simulink model "bench_local_2208"  (R2026a)
settings: Solver=FixedStepDiscrete  StopTime=bench_duration  FixedStep=Ts_plant
model workspace (MAT data in the model file):
  B_load = 0
  B_m = 0.00357610067176
  B_rotor = 1.07e-06
  IQ_LIMIT_MA = 400
  I_console_max_mA = 1800
  Imax = 200
  J_load = 0
  J_m = 5e-07
  J_rotor = 5e-07
  Ke_LL_rms_per_krpm = 7.68
  Ki_i = 0.0008
  Ki_w = 200
  Kp_i = 0.00025
  Kp_w = 27
  L_d = 0.00258
  L_q = 0.00258
  MAX_FILTERED_SPEED = 35
  MAX_PHASE_MA = 800
  MAX_RAW_SPEED = 60
  MOD_LIMIT = 0.12
  R_s = 9.21741944903
  R_shunt = 0.015
  STUCK_CHECK_MOD = 0.02
  STUCK_CHECK_US = 120000
  Ts_ctrl = 0.001
  Ts_plant = 1e-05
  V_dc = 12
  adc_bits = 12
  adc_range_mV = 3100
  alpha_i = 0.15
  alpha_w = 0.05
  b_u_mV = 1680
  b_v_mV = 1680
  bench_amp = 2
  bench_duration = 5
  bench_hz = 1
  bench_speed = 1
  ctrl_dt_max_s = 0.05
  duty_mid = 0.5
  enc_bits = 12
  enc_dt_max_us = 20000
  enc_dt_min_us = 100
  enc_fail_decay = 0.9
  enc_ok = 1
  f_closed_max_Hz = 60
  f_console_max_Hz = 80
  id_target_mA = 0
  load_Nm = 0.002
  mod_limit = 0.4
  motor_x0 = [0; 0; 0; 0]
  ocp_disable_s = 0.02
  ocp_limit_mA = 1500
  ocp_samples = 150
  p_pairs = 7
  psi_pm = 0.00855438776211
  pwm_Hz = 20000
  pwm_bits = 10
  pwm_switching = 0
  restoring_A_per_rad = 1.99244538017
  s_enc = 1
  sense_gain = 50
  sense_sign = -1
  sense_wiring_sign = -1
  sim_end_s = 3
  start_Hz = 0
  start_load_Nm = 0
  step_load_s = 1.25
  step_speed_s = 0.1
  target_Hz = 8
  theta_off = 0
  torque_sign = 1
  unipolar_threshold_mV = 300
Description:
  | BENCH1 small-angle experiment. Model Workspace owns the complete parameter snapshot. R_s (ohm), B_m (N m s/rad), restoring_A_per_rad (A/rad) specify the local plant. Set bench_speed=1 for electrical speed, 0 for q current; bench_hz is the reference frequency and bench_amp is its peak in electrical rad/s or mA.
settings Model: Creator=29113  LastModifiedBy=29113

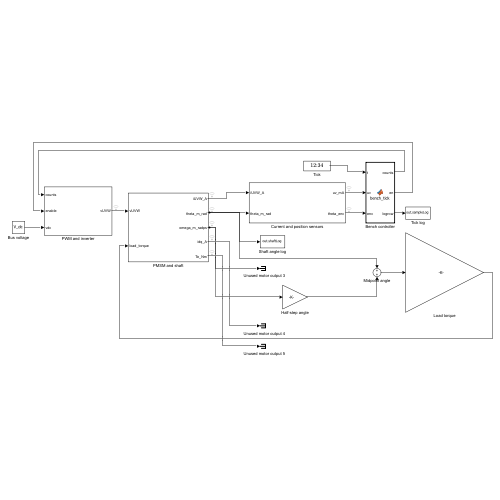
[thumbnail: Simulink's stored preview of the top-level diagram]
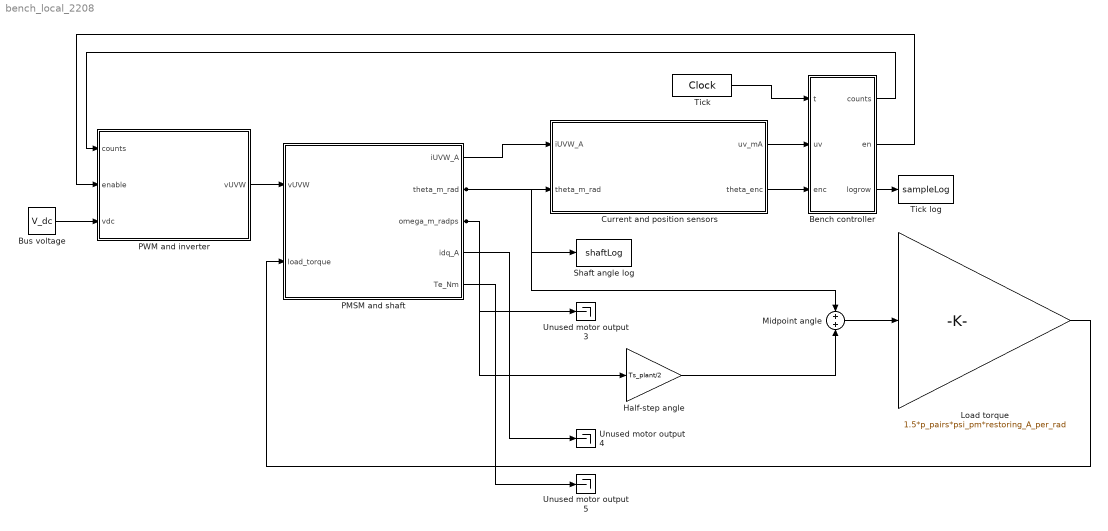
== system bench_local_2208 ==
  Bench controller : MATLAB Function  TreatAsAtomicUnit=on
  Bus voltage : Constant  Value=V_dc  SampleTime=Ts_plant
  Current and position sensors : Subsystem
  Half-step angle : Gain  Gain=Ts_plant/2
  Load torque : Gain  Gain=1.5*p_pairs*psi_pm*restoring_A_per_rad
  Midpoint angle : Sum
  PMSM and shaft : Subsystem
  PWM and inverter : Subsystem
  Shaft angle log : ToWorkspace  VariableName=shaftLog  SaveFormat=Timeseries  SampleTime=Ts_ctrl
  Tick : DigitalClock  SampleTime=Ts_ctrl
  Tick log : ToWorkspace  VariableName=sampleLog  SaveFormat=Timeseries  SampleTime=-1
  Unused motor output 3 : Terminator
  Unused motor output 4 : Terminator
  Unused motor output 5 : Terminator
  wires:
  Bus voltage/1 -> PWM and inverter/3(vdc)
  PMSM and shaft/4(idq_A) -> Unused motor output 4/1
  PWM and inverter/1(vUVW) -> PMSM and shaft/1(vUVW)
  PMSM and shaft/1(iUVW_A) -> Current and position sensors/1(iUVW_A)
  PMSM and shaft/2(theta_m_rad) -> Midpoint angle/1, Current and position sensors/2(theta_m_rad), Shaft angle log/1
  PMSM and shaft/5(Te_Nm) -> Unused motor output 5/1
  PMSM and shaft/3(omega_m_radps) -> Half-step angle/1, Unused motor output 3/1
  Midpoint angle/1 -> Load torque/1
  Tick/1 -> Bench controller/1(t)
  Bench controller/2(en) -> PWM and inverter/2(enable)
  Current and position sensors/1(uv_mA) -> Bench controller/2(uv)
  Current and position sensors/2(theta_enc) -> Bench controller/3(enc)
  Half-step angle/1 -> Midpoint angle/2
  Bench controller/1(counts) -> PWM and inverter/1(counts)
  Bench controller/3(logrow) -> Tick log/1
  Load torque/1 -> PMSM and shaft/2(load_torque)

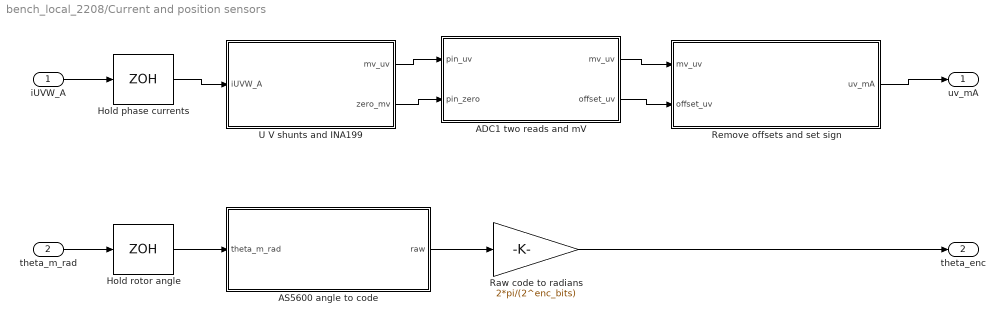
== system bench_local_2208/Current and position sensors ==
  iUVW_A : Inport
  theta_m_rad : Inport  Port=2
  ADC1 two reads and mV : MATLAB Function  TreatAsAtomicUnit=on
  AS5600 angle to code : MATLAB Function  TreatAsAtomicUnit=on
  Hold phase currents : ZeroOrderHold  SampleTime=Ts_ctrl
  Hold rotor angle : ZeroOrderHold  SampleTime=Ts_ctrl
  Raw code to radians : Gain  Gain=2*pi/(2^enc_bits)
  Remove offsets and set sign : MATLAB Function  TreatAsAtomicUnit=on
  U V shunts and INA199 : MATLAB Function  TreatAsAtomicUnit=on
  uv_mA : Outport
  theta_enc : Outport  Port=2
  wires:
  Raw code to radians/1 -> theta_enc/1
  AS5600 angle to code/1(raw) -> Raw code to radians/1
  Hold rotor angle/1 -> AS5600 angle to code/1(theta_m_rad)
  theta_m_rad/1 -> Hold rotor angle/1
  Remove offsets and set sign/1(uv_mA) -> uv_mA/1
  ADC1 two reads and mV/2(offset_uv) -> Remove offsets and set sign/2(offset_uv)
  ADC1 two reads and mV/1(mv_uv) -> Remove offsets and set sign/1(mv_uv)
  U V shunts and INA199/2(zero_mv) -> ADC1 two reads and mV/2(pin_zero)
  U V shunts and INA199/1(mv_uv) -> ADC1 two reads and mV/1(pin_uv)
  Hold phase currents/1 -> U V shunts and INA199/1(iUVW_A)
  iUVW_A/1 -> Hold phase currents/1

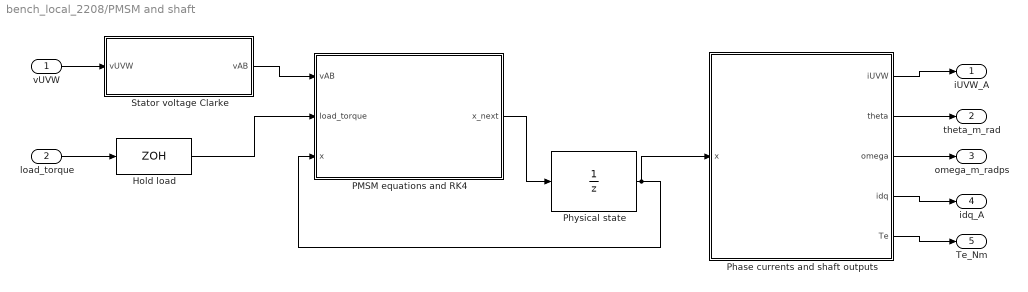
== system bench_local_2208/PMSM and shaft ==
  vUVW : Inport
  load_torque : Inport  Port=2
  Hold load : ZeroOrderHold  SampleTime=Ts_plant
  PMSM equations and RK4 : MATLAB Function  TreatAsAtomicUnit=on
  Phase currents and shaft outputs : MATLAB Function  TreatAsAtomicUnit=on
  Physical state : UnitDelay  InitialCondition=motor_x0  SampleTime=Ts_plant
  Stator voltage Clarke : MATLAB Function  TreatAsAtomicUnit=on
  iUVW_A : Outport
  theta_m_rad : Outport  Port=2
  omega_m_radps : Outport  Port=3
  idq_A : Outport  Port=4
  Te_Nm : Outport  Port=5
  wires:
  PMSM equations and RK4/1(x_next) -> Physical state/1
  Physical state/1 -> Phase currents and shaft outputs/1(x), PMSM equations and RK4/3(x)
  Hold load/1 -> PMSM equations and RK4/2(load_torque)
  load_torque/1 -> Hold load/1
  Stator voltage Clarke/1(vAB) -> PMSM equations and RK4/1(vAB)
  vUVW/1 -> Stator voltage Clarke/1(vUVW)
  Phase currents and shaft outputs/5(Te) -> Te_Nm/1
  Phase currents and shaft outputs/4(idq) -> idq_A/1
  Phase currents and shaft outputs/3(omega) -> omega_m_radps/1
  Phase currents and shaft outputs/2(theta) -> theta_m_rad/1
  Phase currents and shaft outputs/1(iUVW) -> iUVW_A/1

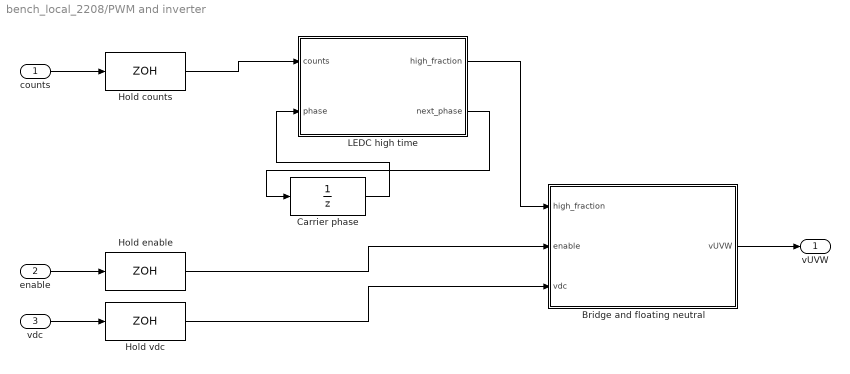
== system bench_local_2208/PWM and inverter ==
  counts : Inport
  enable : Inport  Port=2
  vdc : Inport  Port=3
  Bridge and floating neutral : MATLAB Function  TreatAsAtomicUnit=on
  Carrier phase : UnitDelay  SampleTime=Ts_plant
  Hold counts : ZeroOrderHold  SampleTime=Ts_plant
  Hold enable : ZeroOrderHold  SampleTime=Ts_plant
  Hold vdc : ZeroOrderHold  SampleTime=Ts_plant
  LEDC high time : MATLAB Function  TreatAsAtomicUnit=on
  vUVW : Outport
  wires:
  Bridge and floating neutral/1(vUVW) -> vUVW/1
  Hold vdc/1 -> Bridge and floating neutral/3(vdc)
  Hold enable/1 -> Bridge and floating neutral/2(enable)
  LEDC high time/1(high_fraction) -> Bridge and floating neutral/1(high_fraction)
  LEDC high time/2(next_phase) -> Carrier phase/1
  Carrier phase/1 -> LEDC high time/2(phase)
  Hold counts/1 -> LEDC high time/1(counts)
  vdc/1 -> Hold vdc/1
  enable/1 -> Hold enable/1
  counts/1 -> Hold counts/1

== matlab function bench_local_2208/PMSM and shaft/Phase currents and shaft outputs ==
  data: x input; iUVW output; theta output; omega output; idq output; Te output; p_pairs parameter; L_d parameter; L_q parameter; psi_pm parameter
function [iUVW,theta,omega,idq,Te] = outputs(x, p_pairs, L_d, L_q, psi_pm)
%#codegen
id = x(1); iq = x(2); theta = x(3); omega = x(4);
ct = cos(p_pairs*theta); st = sin(p_pairs*theta);
i_alpha = ct*id - st*iq;
i_beta = st*id + ct*iq;
iUVW = [i_alpha; -.5*i_alpha + sqrt(3)*.5*i_beta; -.5*i_alpha - sqrt(3)*.5*i_beta];
idq = [id; iq];
Te = 1.5*p_pairs*(psi_pm+(L_d-L_q)*id)*iq;
end

== matlab function bench_local_2208/Current and position sensors/U V shunts and INA199 ==
  data: iUVW_A input; mv_uv output; zero_mv output; b_u_mV parameter; b_v_mV parameter; R_shunt parameter; sense_gain parameter; sense_wiring_sign parameter
function [mv_uv, zero_mv] = sense(iUVW_A, b_u_mV, b_v_mV, R_shunt, sense_gain, sense_wiring_sign)
% The physical shunt polarity is independent of the software sign correction.
zero_mv = [b_u_mV; b_v_mV];
amps_uv = [iUVW_A(1); iUVW_A(2)];
mv_uv = zero_mv + sense_wiring_sign * (1000 * R_shunt * sense_gain) * amps_uv;
end

== matlab function bench_local_2208/Current and position sensors/ADC1 two reads and mV ==
  data: pin_uv input; mv_uv output; pin_zero input; offset_uv output; adc_bits parameter; adc_range_mV parameter
function [mv_uv, offset_uv] = adc(pin_uv, pin_zero, adc_bits, adc_range_mV)
% Running samples and the stationary zero calibration use the same ADC model.
last_code = 2^adc_bits - 1;
mv_uv = adc_read_mv(pin_uv, last_code, adc_range_mV);
offset_uv = adc_read_mv(pin_zero, last_code, adc_range_mV);
end
function mv = adc_read_mv(pin_mv, last_code, range_mv)
% The two one-shot reads see the same held voltage. Their integer mean is raw.
clipped_mv = min(max(pin_mv, 0), range_mv);
raw = floor(clipped_mv * (last_code/range_mv) + 0.5);
% main.c:525, without a chip-specific calibration curve.
mv = floor((raw * range_mv) / last_code);
end

== matlab function bench_local_2208/Current and position sensors/Remove offsets and set sign ==
  data: mv_uv input; uv_mA output; offset_uv input; R_shunt parameter; sense_gain parameter; sense_sign parameter; unipolar_threshold_mV parameter
function uv_mA = convert(mv_uv, offset_uv, R_shunt, sense_gain, sense_sign, unipolar_threshold_mV)
% A stationary, disabled motor gives identical readings throughout zero calibration.
delta_mv = mv_uv - offset_uv;
if all(offset_uv < unipolar_threshold_mV)
    delta_mv = max(delta_mv, 0);
end
uv_mA = sense_sign * delta_mv / (R_shunt * sense_gain);
end

== matlab function bench_local_2208/Current and position sensors/AS5600 angle to code ==
  data: theta_m_rad input; raw output; s_enc parameter; p_pairs parameter; theta_off parameter; enc_bits parameter
function raw = encoder(theta_m_rad, s_enc, p_pairs, theta_off, enc_bits)
% Sensor mounting is the inverse of the calibrated mech_to_elec relationship.
angle_rad = mod(s_enc * (theta_m_rad - theta_off / p_pairs), 2*pi);
% Select the angular bin that contains the actual mechanical angle.
bins = 2^enc_bits;
raw = min(bins-1, floor(angle_rad * (bins/(2*pi))));
end

== matlab function bench_local_2208/Bench controller ==
  data: t input; counts output; uv input; enc input; en output; logrow output; bench_speed parameter; bench_amp parameter; bench_hz parameter; bench_duration parameter; Ts_ctrl parameter; p_pairs parameter; s_enc parameter; theta_off parameter; torque_sign parameter; alpha_i parameter; alpha_w parameter; Kp_i parameter; Ki_i parameter; Kp_w parameter; Ki_w parameter; pwm_bits parameter; duty_mid parameter; IQ_LIMIT_MA parameter; MAX_PHASE_MA parameter; MOD_LIMIT parameter; MAX_RAW_SPEED parameter; MAX_FILTERED_SPEED parameter; STUCK_CHECK_MOD parameter; STUCK_CHECK_US parameter
function [counts,en,logrow] = bench_tick(t,uv,enc,bench_speed, bench_amp, ...
bench_hz, bench_duration, Ts_ctrl, p_pairs, s_enc, theta_off, torque_sign, ...
alpha_i, alpha_w, Kp_i, Ki_i, Kp_w, Ki_w, pwm_bits, duty_mid, ...
IQ_LIMIT_MA, MAX_PHASE_MA, MOD_LIMIT, MAX_RAW_SPEED, MAX_FILTERED_SPEED, ...
STUCK_CHECK_MOD, STUCK_CHECK_US)
%#codegen
% BENCH1 starts after calibration with zero PI integrals and zero LPF states.
persistent zd zq zw idf iqf wf prevEnc prevUV flatSince prevMod trip
if isempty(trip)
    zd=0; zq=0; zw=0; idf=0; iqf=0; wf=0;
    prevEnc=enc; prevUV=uv; flatSince=0; prevMod=0; trip=0;
end
levels = 2^pwm_bits-1;
counts = ones(3,1)*floor(duty_mid*levels+0.5);
en = 0;
ref = bench_amp*sin(2*pi*bench_hz*t);
logrow = [ref;0;0;0;0;0;trip];
if t<=0 || t>=bench_duration || trip~=0, return; end
if max(abs([uv(1);uv(2);-sum(uv)]))>=MAX_PHASE_MA
    trip=1;
elseif prevMod<STUCK_CHECK_MOD || any(uv~=prevUV)
    flatSince=t;
elseif (t-flatSince)*1e6>=STUCK_CHECK_US
    trip=4;
end
prevUV=uv;
delta = mod(enc-prevEnc+pi,2*pi)-pi;
raw = p_pairs*delta/Ts_ctrl;
prevEnc=enc;
if trip==0
    if abs(raw)>MAX_RAW_SPEED
        trip=2;
    else
        wf=wf+alpha_w*(raw-wf);
        if abs(wf)>MAX_FILTERED_SPEED, trip=3; end
    end
end
if trip~=0, logrow(7)=trip; return; end
theta=s_enc*p_pairs*enc+theta_off+wf*Ts_ctrl;
c=cos(theta); sn=sin(theta); beta=(uv(1)+2*uv(2))/sqrt(3);
id=uv(1)*c+beta*sn; iq=-uv(1)*sn+beta*c;
idf=idf+alpha_i*(id-idf); iqf=iqf+alpha_i*(iq-iqf);
target=ref; speedLimited=false;
if bench_speed~=0
    [target,zw,speedLimited]=pi_step(zw,ref-wf,Kp_w,Ki_w,Ts_ctrl,IQ_LIMIT_MA);
    target=torque_sign*s_enc*target;
end
[d,zd,dLimited]=pi_step(zd,-idf,Kp_i,Ki_i,Ts_ctrl,MOD_LIMIT);
[q,zq,qLimited]=pi_step(zq,target-iqf,Kp_i,Ki_i,Ts_ctrl,MOD_LIMIT);
mag=hypot(d,q);
if mag>MOD_LIMIT, d=d*MOD_LIMIT/mag; q=q*MOD_LIMIT/mag; end
prevMod=min(mag,MOD_LIMIT);
a=d*c-q*sn; b=d*sn+q*c;
phases=[a; -0.5*a+sqrt(3)*0.5*b; -0.5*a-sqrt(3)*0.5*b];
counts=floor((duty_mid+phases)*levels+0.5);
en=1;
logrow=[ref;iq;iqf;raw;wf;double(speedLimited || dLimited || qLimited || mag>MOD_LIMIT);trip];
end

function [u,next,limited]=pi_step(x,error,kp,ki,dt,limit)
cmd=x+kp*error;
limited=abs(cmd)>limit;
next=x;
if ~limited || cmd*error<0, next=min(limit,max(-limit,x+ki*dt*error)); end
u=min(limit,max(-limit,cmd));
end

== matlab function bench_local_2208/PWM and inverter/LEDC high time ==
  data: counts input; high_fraction output; phase input; next_phase output; Ts_plant parameter; pwm_switching parameter; pwm_Hz parameter; pwm_bits parameter
function [high_fraction, next_phase] = pwm_interval(counts, phase, Ts_plant, pwm_switching, pwm_Hz, pwm_bits)
%#codegen
% The hardware counter has 2^pwm_bits states, with a high fraction of N/levels.
% The interval starts at the stored leading-edge carrier phase.
levels = 2^pwm_bits;
periods = pwm_Hz * Ts_plant;
stop = phase + periods;
next_phase = mod(stop,1);
high_fraction = zeros(3,1);
for k = 1:3
    duty = min(levels-1,max(0,round(counts(k)))) / levels;
    if pwm_switching ~= 0
        % Integral of the rectangular pulse train, in carrier periods.
        start_area = min(phase,duty);
        stop_area = floor(stop)*duty + min(mod(stop,1),duty);
        high_fraction(k) = min(1,max(0,(stop_area-start_area)/periods));
    else
        high_fraction(k) = duty;
    end
end
end

== matlab function bench_local_2208/PWM and inverter/Bridge and floating neutral ==
  data: high_fraction input; vUVW output; enable input; vdc input
function vUVW = bridge_voltage(high_fraction, enable, vdc)
%#codegen
% An ideal two-level bridge feeding a balanced three-wire star.
vUVW = zeros(3,1);
if enable ~= 0
    v_pole = vdc * high_fraction;
    v_neutral = (v_pole(1) + v_pole(2) + v_pole(3)) / 3;
    vUVW = v_pole - v_neutral;
end
% Disabled approximation: equal pole potentials, zero line-line voltages.
end

== matlab function bench_local_2208/PMSM and shaft/Stator voltage Clarke ==
  data: vUVW input; vAB output
function vAB = stator_voltage(vUVW)
%#codegen
% Amplitude-invariant Clarke transform; common mode cancels.
vAB = [(2*vUVW(1)-vUVW(2)-vUVW(3))/3; (vUVW(2)-vUVW(3))/sqrt(3)];
end

== matlab function bench_local_2208/PMSM and shaft/PMSM equations and RK4 ==
  data: vAB input; x_next output; load_torque input; x input; Ts_plant parameter; p_pairs parameter; R_s parameter; L_d parameter; L_q parameter; psi_pm parameter; J_m parameter; B_m parameter
function x_next = advance_pmsm(vAB, load_torque, x, Ts_plant, p_pairs, R_s, L_d, L_q, psi_pm, J_m, B_m)
%#codegen
% x = [id (A); iq (A); mechanical angle (rad); mechanical speed (rad/s)].
% Hold stationary-frame voltage and load over the integration interval.
h = Ts_plant;
k1 = derivative(x,vAB,load_torque,p_pairs,R_s,L_d,L_q,psi_pm,J_m,B_m);
k2 = derivative(x+h*k1/2,vAB,load_torque,p_pairs,R_s,L_d,L_q,psi_pm,J_m,B_m);
k3 = derivative(x+h*k2/2,vAB,load_torque,p_pairs,R_s,L_d,L_q,psi_pm,J_m,B_m);
k4 = derivative(x+h*k3,vAB,load_torque,p_pairs,R_s,L_d,L_q,psi_pm,J_m,B_m);
x_next = x + (h/6)*(k1+2*k2+2*k3+k4);
end

function dx = derivative(x,vAB,load_torque,p,R,Ld,Lq,psi,J,B)
id = x(1); iq = x(2); theta = x(3); omega = x(4);
ct = cos(p*theta); st = sin(p*theta);
vd =  ct*vAB(1) + st*vAB(2);
vq = -st*vAB(1) + ct*vAB(2);
we = p*omega;
did = (vd - R*id + we*Lq*iq)/Ld;
diq = (vq - R*iq - we*(Ld*id + psi))/Lq;
Te = 1.5*p*(psi + (Ld-Lq)*id)*iq;
dx = [did; diq; omega; (Te - load_torque - B*omega)/J];
end
